simulink model "sf_bind_fcn_call_subsys_muxed_triggers"  (R2025b)
settings: Solver=FixedStepDiscrete  StartTime=0.0  StopTime=22  FixedStep=1  RelTol=1e-3  EnableMultiTasking=on
settings Model: Creator=The MathWorks, Inc.  LastModifiedBy=The MathWorks, Inc.
settings SolverCC: AlgebraicLoopSolver=TrustRegion
settings DataIOCC: LimitDataPoints=on  SaveFormat=Array  ReturnWorkspaceOutputs=off  SignalLoggingName=sigsOut
settings OptimizationCC: ReuseModelBlockBuffer=off  ExpressionDepthLimit=2147483647.0  InitFltsAndDblsToZero=on  LifeSpan=inf
settings DebuggingCC: SaveWithParameterizedLinksMsg=none  UnderspecifiedInitializationDetection=Classic  MergeDetectMultiDrivingBlocksExec=none  CheckExecutionContextPreStartOutputMsg=on  MultiTaskDSMMsg=warning  MultiTaskCondExecSysMsg=none  FcnCallInpInsideContextMsg=warning  UnconnectedInputMsg=warning  UnconnectedOutputMsg=warning  UnconnectedLineMsg=warning  StateNameClashWarn=warning  SFUnexpectedBacktrackingDiag=warning  SFNoUnconditionalDefaultTransitionDiag=warning  SFExecutionAtInitializationDiag=none  ArithmeticOperatorsInVariantConditions=warning
settings HardwareCC: ProdBitPerPointer=32.0  ProdBitPerSizeT=32.0  ProdBitPerPtrDiffT=32.0  ProdLargestAtomicFloat=None  ProdIntDivRoundTo=Undefined  ProdEndianess=Unspecified  ProdWordSize=32.0  ProdHWDeviceType=32-bit Generic  TargetUnknown=on
settings ModelReferenceCC: UpdateModelReferenceTargets=IfOutOfDate  EnableRefExpFcnMdlSchedulingChecks=on  PropagateSignalLabelsOutOfModel=off
settings SFSimCC: SimUseLocalCustomCode=off  SimParseCustomCode=off  CustomCodeUndefinedFunction=UseInterfaceOnly
settings RTWCC: RTWUseLocalCustomCode=off  GPUComputeCapability=3.5  DLArmComputeVersion=19.05
settings CodeAppCC: StateflowObjectComments=on
settings GRTTargetCC: TargetFcnLib=ansi_tfl_tmw.mat  TargetLangStandard=C89/C90 (ANSI)  CombineOutputUpdateFcns=off  GRTInterface=on
settings ConfigComp: CovMetricSettings=dw  CovSaveCumulativeToWorkspaceVar=on  CovSaveSingleToWorkspaceVar=on  CovExternalEMLEnable=off

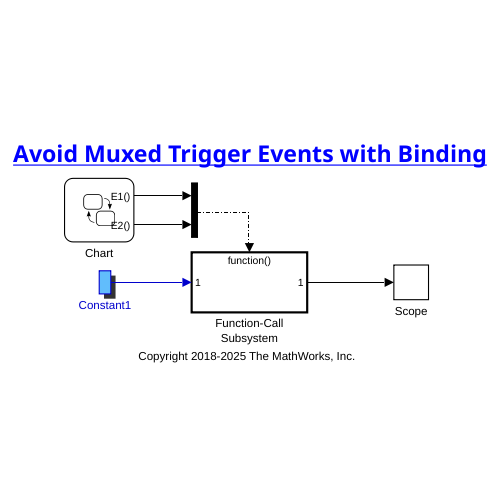
[thumbnail: Simulink's stored preview of the top-level diagram]
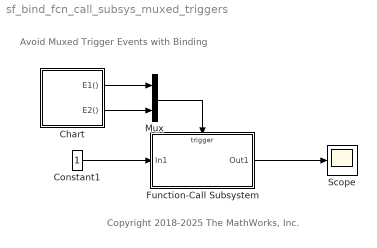
== system sf_bind_fcn_call_subsys_muxed_triggers ==
  note: Copyright 2018-2025 The MathWorks, Inc.
  note: Avoid Muxed Trigger Events with Binding
  Chart : Stateflow chart  TreatAsAtomicUnit=on
  Constant1 : Constant
  Function-Call Subsystem : Subsystem  TreatAsAtomicUnit=on
  Mux : Mux  Inputs=2
  Scope : Scope
      settings: ActiveDisplayYMaximum=25
  wires:
  Constant1/1 -> Function-Call Subsystem/1(In1)
  Function-Call Subsystem/1(Out1) -> Scope/1
  Chart/1(E1()) -> Mux/1
  Chart/2(E2()) -> Mux/2
  Mux/1 -> Function-Call Subsystem/Trigger

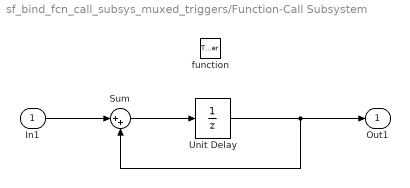
== system sf_bind_fcn_call_subsys_muxed_triggers/Function-Call Subsystem ==
  In1 : Inport
  function : TriggerPort  TriggerType=function-call  VariantControl=Variant  StatesWhenEnabling=reset
  Sum : Sum  Inputs=|++  InputSameDT=on  SaturateOnIntegerOverflow=on  OutDataTypeStr=Inherit: Same as first input
  Unit Delay : UnitDelay  SampleTime=-1  HasFrameUpgradeWarning=on
  Out1 : Outport  OutputWhenDisabled=reset  InitialOutput=0  VectorParamsAs1DForOutWhenUnconnected=off
  wires:
  In1/1 -> Sum/1
  Sum/1 -> Unit Delay/1
  Unit Delay/1 -> Out1/1, Sum/2

== stateflow chart sf_bind_fcn_call_subsys_muxed_triggers/Chart ==
  state A1
    bind: E1;
    en,du: E1;
  state B1
    en: E2;
  (default) -> A1
  A1 -> B1 : after(10,tick)
  B1 -> A1
  events: E1 output FUNCTION_CALL_EVENT; E2 output FUNCTION_CALL_EVENT
